simulink model "Photovoltaic_Model03"  (R2026a)
settings: Solver=VariableStepAuto  StopTime=10
values from neighbouring files (symbols this model uses):
  G = prueba (i)    [CurvasPhotovoltaic_M25290062.m]
  Rsh = 415.405    [CurvasPhotovoltaic_M25290062.m]
  T = 25    [CurvasPhotovoltaic_M25290062.m]
libraries: simulink x1
settings Model: Creator=Usuario  LastModifiedBy=carloschavez

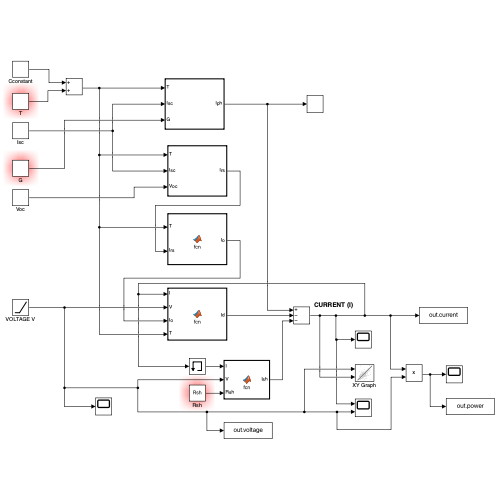
[thumbnail: Simulink's stored preview of the top-level diagram]
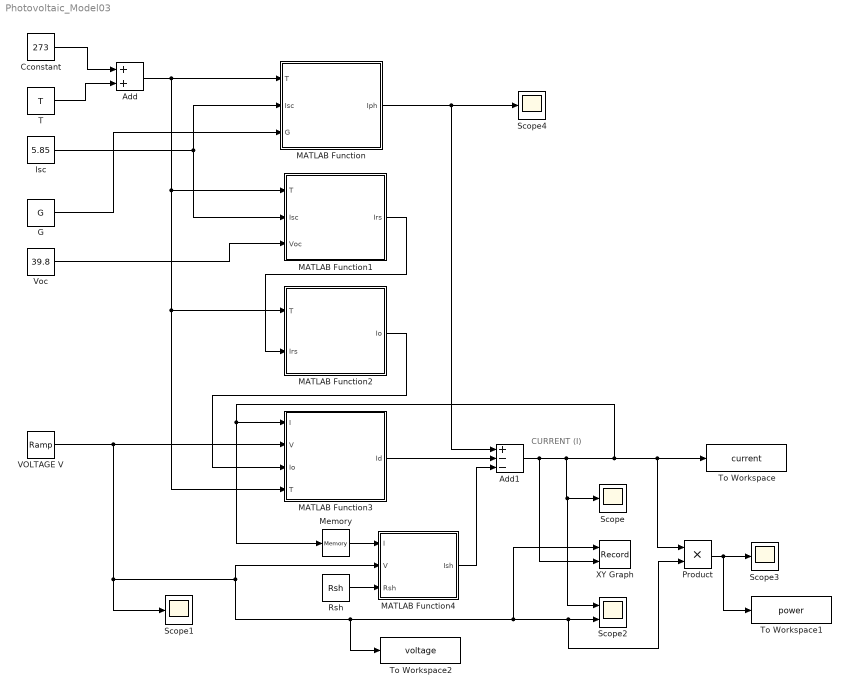
== system Photovoltaic_Model03 ==
  note: CURRENT (I)
  Add : Sum
  Add1 : Sum  Inputs=+--
  Cconstant : Constant  Value=273
  G : Constant  Value=G
  Isc : Constant  Value=5.85
  MATLAB Function : MATLAB Function  TreatAsAtomicUnit=on
  MATLAB Function1 : MATLAB Function  TreatAsAtomicUnit=on
  MATLAB Function2 : MATLAB Function  TreatAsAtomicUnit=on
  MATLAB Function3 : MATLAB Function  TreatAsAtomicUnit=on
  MATLAB Function4 : MATLAB Function  TreatAsAtomicUnit=on
  Memory : Memory
  Product : Product
  Rsh : Constant  Value=Rsh
  Scope{,1,3..4} (4 alike) : Scope
      Scope settings: ActiveDisplayYMinimum=-9.97604478916195  ActiveDisplayYMaximum=8.3217392457172537
      Scope1 settings: ActiveDisplayYMinimum=-1  ActiveDisplayYMaximum=1
      Scope3 settings: ActiveDisplayYMinimum=-1  ActiveDisplayYMaximum=1
      Scope4 settings: ActiveDisplayYMinimum=-1  ActiveDisplayYMaximum=1  DataLoggingVariableName=ScopeData3
  Scope2 : Scope  NumInputPorts=2
      settings: ActiveDisplayYMinimum=-1  ActiveDisplayYMaximum=1  DataLoggingVariableName=ScopeData2
  T : Constant  Value=T
  To Workspace : ToWorkspace  VariableName=current  SampleTime=-1
  To Workspace1 : ToWorkspace  VariableName=power  SampleTime=-1
  To Workspace2 : ToWorkspace  VariableName=voltage  SampleTime=-1
  VOLTAGE V : simulink/Sources/Ramp  slope=4.5  start=0  InitialOutput=0
  Voc : Constant  Value=39.8
  XY Graph : Record  NumPorts=2.0  FileSettingsInternal="{\"entries\":[{\"content\":{\"excelSettings\":{\"content\":{},\"type\":\"Streamout.ExcelSettings\"},\"parquetSettings\":{\"content\":{},\"type\":\"Streamout.ParquetSettings\"}},\"type\":\"Streamout.FileSettingStorage\",\"uuid\":\"\"}],\"packageUris\":[\"http:\\/\\/schema.mathworks.com\\/mf0\\/streamout_blocks\\/R2020a\"],\"version\":\"1.0\"}"  FrameSettings=[0, 0]  Layout=[1 1]  SignalsInternal="{\"entries\":[{\"content\":{\"signals\":[{\"content\":{\"blockPath\":[],\"dimensions\":[1],\"domain\":\"\",\"lineColor\":\"#a2142f\",\"plots\":[ 1 ],\"port\":1,\"signalID\":1,\"signalName\":\"VOLTAGE V\"},\"type\":\"RecordBlkView.Signal\",\"uuid\":\"\"},{\"content\":{\"blockPath\":[],\"dimensions\":[1],\"domain\":\"\",\"lineColor\":\"#139fff\",\"plots\":[ 1 ],\"port\":2,\"signalID\":2,\"signalName\":\"Add1\"},\"type\":\"RecordBlkView.Signal\",\"uuid\":\"\"}]},\"type\":\"RecordBlkView.InputSignals\",\"uuid\":\"\"}],\"packageUris\":[\"http:\\/\\/schema.mathworks.com\\/mf0\\/streamout_blocks\\/R2020a\"],\"version\":\"1.0\"}"  VisualizationBindings="{\"xyplotplugin\":{\"info\":[{\"series\":[{\"bindingParametersList\":[{\"parameter\":\"X-Axis\",\"signalID\":1,\"signalName\":\"VOLTAGE V\"},{\"parameter\":\"Y-Axis\",\"signalID\":2,\"signalName\":\"Add1\"}],\"seriesID\":0}],\"subplotID\":1}]}}"  CompatibilityTag=XY
  wires:
  Cconstant/1 -> Add/1
  T/1 -> Add/2
  Add/1 -> MATLAB Function3/4(T), MATLAB Function2/1(T), MATLAB Function1/1(T), MATLAB Function/1(T)
  MATLAB Function1/1(Irs) -> MATLAB Function2/2(Irs)
  Isc/1 -> MATLAB Function/2(Isc), MATLAB Function1/2(Isc)
  G/1 -> MATLAB Function/3(G)
  Voc/1 -> MATLAB Function1/3(Voc)
  MATLAB Function2/1(Io) -> MATLAB Function3/3(Io)
  VOLTAGE V/1 -> Scope1/1, MATLAB Function4/2(V), To Workspace2/1, XY Graph/1, Product/2, Scope2/2, MATLAB Function3/2(V)
  MATLAB Function/1(Iph) -> Scope4/1, Add1/1
  MATLAB Function3/1(Id) -> Add1/2
  MATLAB Function4/1(Ish) -> Add1/3
  Add1/1 -> XY Graph/2, Scope2/1, Scope/1, To Workspace/1, Product/1, Memory/1, MATLAB Function3/1(I)
  Product/1 -> To Workspace1/1, Scope3/1
  Rsh/1 -> MATLAB Function4/3(Rsh)
  Memory/1 -> MATLAB Function4/1(I)

== matlab function Photovoltaic_Model03/MATLAB Function1 ==
  data: T input; Irs output; Isc input; Voc input
function Irs = fcn(T, Isc, Voc)

q = 1.6e-19;    %Electron charge (q)
n = 1.3;        %Idealty factor
k = 1.38e-23;   %Boltzmann's Constant (k)
Ns = 54;        %Number of cells conected in series (Ns)

argden = exp((q*Voc)/(n*k*T*Ns))-1;
Irs = Isc / argden ;

== matlab function Photovoltaic_Model03/MATLAB Function ==
  data: T input; Iph output; Isc input; G input
function Iph = fcn(T, Isc, G)

Ki = 0.0032;                          % Short Circuit Current at cell Ki in Amperes.
Iph = (Isc + Ki*(T-298))*(G/1000);

== matlab function Photovoltaic_Model03/MATLAB Function2 ==
  data: T input; Io output; Irs input
function Io = fcn(T, Irs)

Tn = 298;       %Nominal Temperature (Tn)
q = 1.6e-19;    %Electron charge (q)
n = 1.3;        %Idealty factor (n)
k = 1.38e-23;   %Boltzmann's Constant (k)
Ego = 1.1;      %Bandgap Energy (Ego)

Io = (Irs*(T/Tn)^3)*exp(q*Ego*((1/Tn)-(1/T))*(1/(n*k)));

== matlab function Photovoltaic_Model03/MATLAB Function3 ==
  data: I input; V input; Io input; T input; Id output
function Id = fcn(I, V, Io, T)

q = 1.6e-19;    %Electron charge (q)
n = 1.3;        %Idealty factor (n)
k = 1.38e-23;   %Boltzmann's Constant (k)
Rs = 0.221;     %Series Resistance (Rs)
Ns = 54;        %Number of cells conected in series (Ns)

arg_num = q*(V+I*Rs);
arg_den = n*k*T*Ns;

Id = Io*(exp(arg_num/arg_den)-1);

== matlab function Photovoltaic_Model03/MATLAB Function4 ==
  data: I input; Ish output; V input; Rsh input
function Ish = fcn(I, V, Rsh)

Rs = 0.221;  %Series Resistance

Ish = (V+I*Rs)/Rsh;   %Shunt Current
